simulink library "sensorsLibrary"  (R2026a)
settings: Solver=ode45  EnableMultiTasking=on
undefined symbols (not defined in the file): Sensors
libraries: aerolibnav x1
settings Model: Creator=The MathWorks, Inc.  LastModifiedBy=The MathWorks, Inc.
settings DebuggingCC: SymbolicDimsDataTypeCodeGenerationDiagnostic=none
settings HardwareCC: ProdHWDeviceType=32-bit Generic

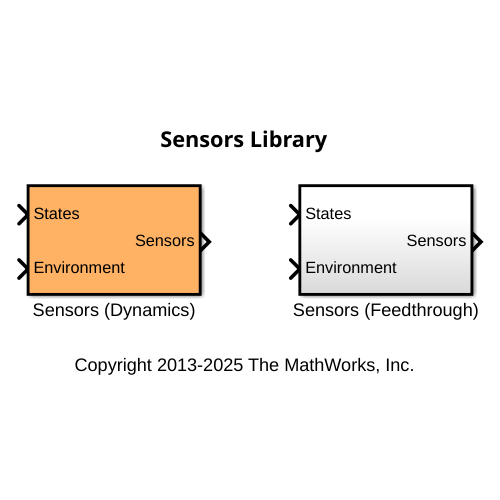
[thumbnail: Simulink's stored preview of the top-level diagram]
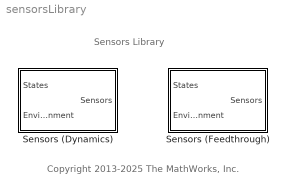
== system sensorsLibrary ==
  note: Copyright 2013-2025 The MathWorks, Inc.
  note: Sensors Library
  Sensors (Dynamics) : Subsystem  TreatAsAtomicUnit=on  VariantControl=Variants.Sensors==1
      mask init:
      | sensorsDynamicsVars;
  Sensors (Feedthrough) : Subsystem  TreatAsAtomicUnit=on

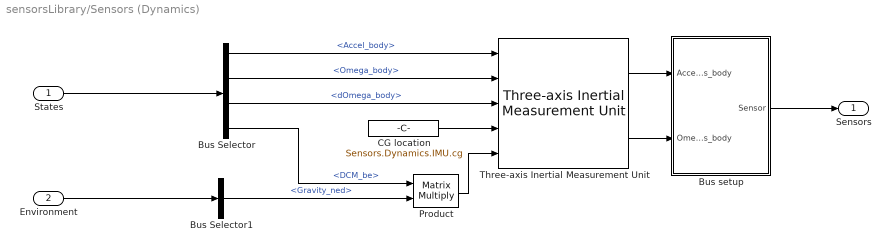
== system sensorsLibrary/Sensors (Dynamics) ==
  States : Inport  OutDataTypeStr=Bus: StatesBus
  Environment : Inport  Port=2  OutDataTypeStr=Bus: EnvironmentBus
  Bus Selector : BusSelector  OutputSignals=Accel_body,Omega_body,dOmega_body,DCM_be
  Bus Selector1 : BusSelector  OutputSignals=Gravity_ned
  Bus setup : Subsystem
  CG location : Constant  Value=Sensors.Dynamics.IMU.cg
  Product : Product  Multiplication=Matrix(*)
  Three-axis Inertial Measurement Unit : aerolibnav/Three-axis Inertial Measurement Unit  units=Metric (MKS)  imu=Sensors.Dynamics.IMU.imu  i_Ts=Ts  dtype_a=on  w_a=Sensors.Dynamics.IMU.accNatFreq  z_a=Sensors.Dynamics.IMU.accDamping  a_sf_cc=Sensors.Dynamics.IMU.accScaleCross  a_bias=Sensors.Dynamics.IMU.accBias  a_sat=Sensors.Dynamics.IMU.accLimits  dtype_g=on  w_g=Sensors.Dynamics.IMU.gyroNatFreq  z_g=Sensors.Dynamics.IMU.gyroDamping  g_sf_cc=Sensors.Dynamics.IMU.gyroScaleCross  g_bias=Sensors.Dynamics.IMU.gyroBias  g_sens=Sensors.Dynamics.IMU.gyroGBias  g_sat=Sensors.Dynamics.IMU.gyroLimits  i_rand=on  i_seeds=Sensors.Dynamics.IMU.noiseSeeds  i_pow=Sensors.Dynamics.IMU.noisePower
  Sensors : Outport  OutDataTypeStr=Bus: SensorsBus  VectorParamsAs1DForOutWhenUnconnected=off
  wires:
  Bus Selector/1 -> Three-axis Inertial Measurement Unit/1  "<Accel_body>"
  Bus Selector/2 -> Three-axis Inertial Measurement Unit/2  "<Omega_body>"
  Environment/1 -> Bus Selector1/1
  Bus Selector/3 -> Three-axis Inertial Measurement Unit/3  "<dOmega_body>"
  CG location/1 -> Three-axis Inertial Measurement Unit/4
  Bus Selector/4 -> Product/1  "<DCM_be>"
  Bus setup/1(Sensor) -> Sensors/1
  Bus Selector1/1 -> Product/2  "<Gravity_ned>"
  Product/1 -> Three-axis Inertial Measurement Unit/5
  Three-axis Inertial Measurement Unit/1 -> Bus setup/1(AccelMeas_body)
  Three-axis Inertial Measurement Unit/2 -> Bus setup/2(OmegaMeas_body)
  States/1 -> Bus Selector/1

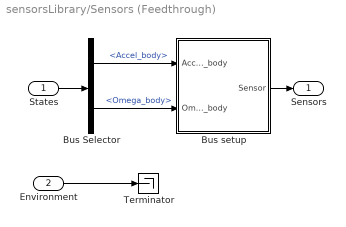
== system sensorsLibrary/Sensors (Feedthrough) ==
  States : Inport  OutDataTypeStr=Bus: StatesBus
  Environment : Inport  Port=2  OutDataTypeStr=Bus: EnvironmentBus
  Bus Selector : BusSelector  OutputSignals=Accel_body,Omega_body
  Bus setup : Subsystem
  Terminator : Terminator
  Sensors : Outport  OutDataTypeStr=Bus: SensorsBus  VectorParamsAs1DForOutWhenUnconnected=off
  wires:
  States/1 -> Bus Selector/1
  Bus setup/1(Sensor) -> Sensors/1
  Bus Selector/2 -> Bus setup/2(OmegaMeas_body)  "<Omega_body>"
  Bus Selector/1 -> Bus setup/1(AccelMeas_body)  "<Accel_body>"
  Environment/1 -> Terminator/1

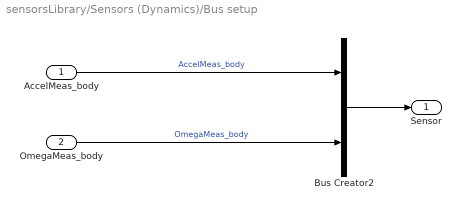
== system sensorsLibrary/Sensors (Dynamics)/Bus setup ==
  AccelMeas_body : Inport
  OmegaMeas_body : Inport  Port=2
  Bus Creator2 : BusCreator  Inputs=2  OutDataTypeStr=Bus: SensorsBus  NonVirtualBus=on
  Sensor : Outport  OutDataTypeStr=Bus: SensorsBus  VectorParamsAs1DForOutWhenUnconnected=off
  wires:
  AccelMeas_body/1 -> Bus Creator2/1  "AccelMeas_body"
  OmegaMeas_body/1 -> Bus Creator2/2  "OmegaMeas_body"
  Bus Creator2/1 -> Sensor/1

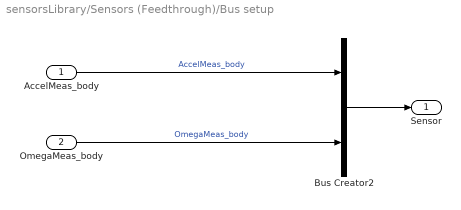
== system sensorsLibrary/Sensors (Feedthrough)/Bus setup ==
  AccelMeas_body : Inport
  OmegaMeas_body : Inport  Port=2
  Bus Creator2 : BusCreator  Inputs=2  OutDataTypeStr=Bus: SensorsBus  NonVirtualBus=on
  Sensor : Outport  OutDataTypeStr=Bus: SensorsBus  VectorParamsAs1DForOutWhenUnconnected=off
  wires:
  AccelMeas_body/1 -> Bus Creator2/1  "AccelMeas_body"
  OmegaMeas_body/1 -> Bus Creator2/2  "OmegaMeas_body"
  Bus Creator2/1 -> Sensor/1
